simulink model "dc_motor_mpc"  (R2025b)
settings: Solver=ode45  StartTime=0.0  StopTime=10  MaxStep=0.001  RelTol=1e-7  AbsTol=1e-9
InitFcn:
  | load(fullfile(fileparts(get_param(bdroot,'FileName')),'dc_motor_mpc_controller.mat'));
model workspace (MAT data in the model file):
  J = 0.01
  Ke = 0.1
  Kt = 0.1
  L = 0.01
  R = 1
  b = 0.001
libraries: mpclib x1
settings Model: Creator=alosw  LastModifiedBy=alosw

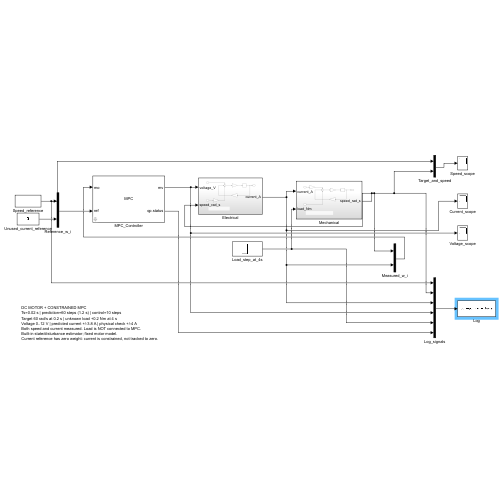
[thumbnail: Simulink's stored preview of the top-level diagram]
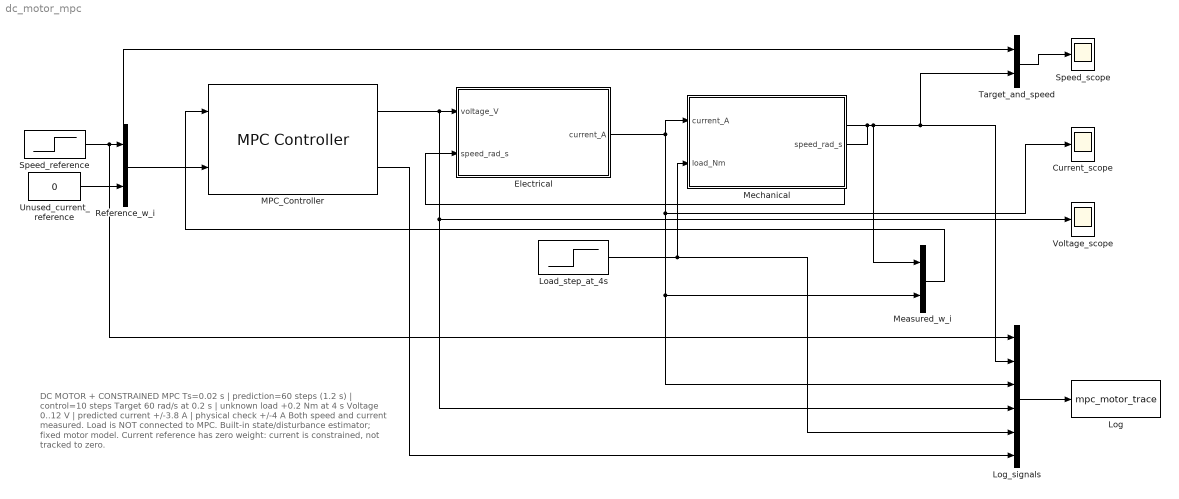
== system dc_motor_mpc ==
  note: DC MOTOR + CONSTRAINED MPC
      | Ts=0.02 s | prediction=60 steps (1.2 s) | control=10 steps
      | Target 60 rad/s at 0.2 s | unknown load +0.2 Nm at 4 s
      | Voltage 0..12 V | predicted current +/-3.8 A | physical check +/-4 A
      | Both speed and current measured. Load is NOT connected to MPC.
      | Built-in state/disturbance estimator; fixed motor model.
      | Current reference has zero weight: current is constrained, not tracked to zero.
  Current_scope : Scope
      settings: ActiveDisplayYMinimum=0.39220982248527481  ActiveDisplayYMaximum=5.1647461781132824
  Electrical : Subsystem
  Load_step_at_4s : Step  Time=4  After=0.2  SampleTime=0
  Log : ToWorkspace  VariableName=mpc_motor_trace  SaveFormat=Timeseries  SampleTime=-1
  Log_signals : Mux  Inputs=6
  MPC_Controller : mpclib/MPC Controller  SCDEnableBlockLinearizationSpecification=on  mpcobj=dc_motor_mpc_controller  is_multiple=0  enable_value=0  return_u0=off  updateMPCinCallerWorkspace=on  md_inport=off  mv_inport=off  uref_inport=off  return_cost=off  return_mvseq=off  return_qpstatus=on  return_xseq=off  return_state=off  return_ovseq=off  state_inport=off  umin_inport=off  umax_inport=off  ymin_inport=off  ymax_inport=off  cc_inport=off  ywt_inport=off  uwt_inport=off  duwt_inport=off  rhoeps_inport=off  pm_inport=off  MaximumP=10  HorizonChoice=FixedHorizon  n_ts=0.02  n_p=60  n_mv=1  n_md=0  n_ud=1  n_mo=2  n_uo=0  BlockDataType=double  SampleTimeInherited=off  switch_inport=off
  Measured_w_i : Mux  Inputs=2
  Mechanical : Subsystem
  Reference_w_i : Mux  Inputs=2
  Speed_reference : Step  Time=0.2  After=60  SampleTime=0
  Speed_scope : Scope
      settings: ActiveDisplayYMinimum=11.383484207123125  ActiveDisplayYMaximum=76.3645095203421
  Target_and_speed : Mux  Inputs=2
  Unused_current_reference : Constant  Value=0
  Voltage_scope : Scope
      settings: ActiveDisplayYMinimum=-1.2061546658932489  ActiveDisplayYMaximum=10.855391993039243
  wires:
  Speed_reference/1 -> Reference_w_i/1, Target_and_speed/1, Log_signals/1
  Unused_current_reference/1 -> Reference_w_i/2
  Reference_w_i/1 -> MPC_Controller/2
  Measured_w_i/1 -> MPC_Controller/1
  MPC_Controller/1 -> Voltage_scope/1, Log_signals/4, Electrical/1(voltage_V)
  Electrical/1(current_A) -> Mechanical/1(current_A), Measured_w_i/2, Log_signals/3, Current_scope/1
  Mechanical/1(speed_rad_s) -> Electrical/2(speed_rad_s), Target_and_speed/2, Log_signals/2, Measured_w_i/1
  Load_step_at_4s/1 -> Mechanical/2(load_Nm), Log_signals/5
  Target_and_speed/1 -> Speed_scope/1
  MPC_Controller/2 -> Log_signals/6
  Log_signals/1 -> Log/1

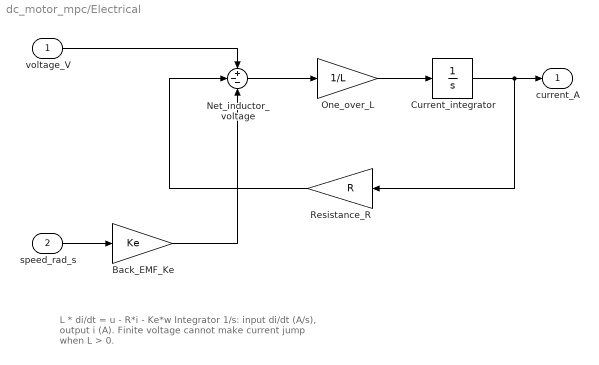
== system dc_motor_mpc/Electrical ==
  note: L * di/dt = u - R*i - Ke*w
      | Integrator 1/s: input di/dt (A/s), output i (A).
      | Finite voltage cannot make current jump when L > 0.
  voltage_V : Inport
  speed_rad_s : Inport  Port=2
  Back_EMF_Ke : Gain  Gain=Ke
  Current_integrator : Integrator
  Net_inductor_voltage : Sum  Inputs=+--
  One_over_L : Gain  Gain=1/L
  Resistance_R : Gain  Gain=R
  current_A : Outport
  wires:
  speed_rad_s/1 -> Back_EMF_Ke/1
  Current_integrator/1 -> Resistance_R/1, current_A/1
  One_over_L/1 -> Current_integrator/1
  Net_inductor_voltage/1 -> One_over_L/1
  Back_EMF_Ke/1 -> Net_inductor_voltage/3
  Resistance_R/1 -> Net_inductor_voltage/2
  voltage_V/1 -> Net_inductor_voltage/1

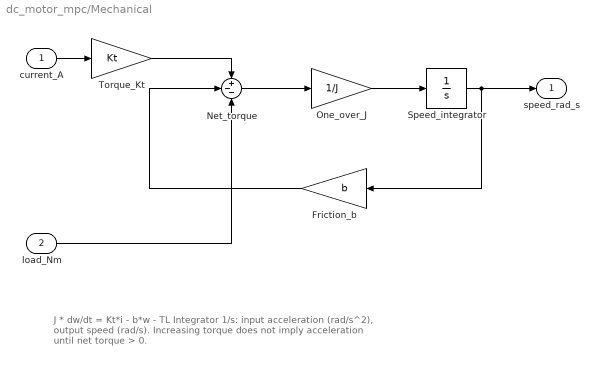
== system dc_motor_mpc/Mechanical ==
  note: J * dw/dt = Kt*i - b*w - TL
      | Integrator 1/s: input acceleration (rad/s^2), output speed (rad/s).
      | Increasing torque does not imply acceleration until net torque > 0.
  current_A : Inport
  load_Nm : Inport  Port=2
  Friction_b : Gain  Gain=b
  Net_torque : Sum  Inputs=+--
  One_over_J : Gain  Gain=1/J
  Speed_integrator : Integrator
  Torque_Kt : Gain  Gain=Kt
  speed_rad_s : Outport
  wires:
  Speed_integrator/1 -> Friction_b/1, speed_rad_s/1
  One_over_J/1 -> Speed_integrator/1
  Net_torque/1 -> One_over_J/1
  load_Nm/1 -> Net_torque/3
  Friction_b/1 -> Net_torque/2
  Torque_Kt/1 -> Net_torque/1
  current_A/1 -> Torque_Kt/1
